simulink model "scheme_L2"  (R2025a)
settings: Solver=ode45  StartTime=0.0  StopTime=12  MaxStep=0.005  RelTol=1e-9  AbsTol=1e-11
settings Model: Creator=dmitriy-nkv  LastModifiedBy=dmitriy-nkv

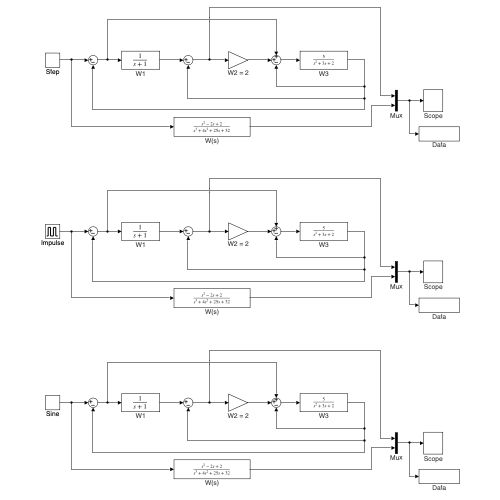
[thumbnail: Simulink's stored preview of the top-level diagram]
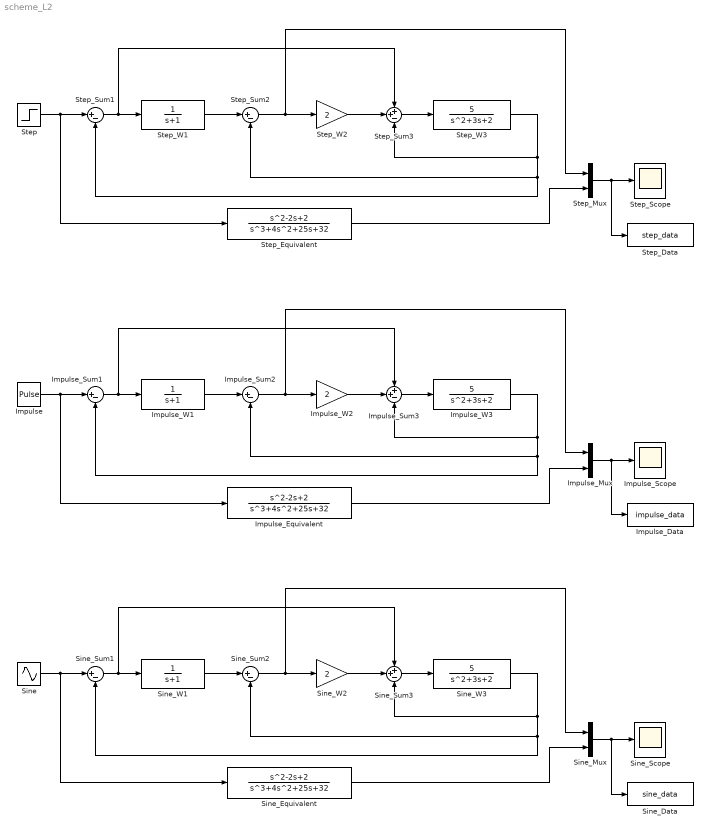
== system scheme_L2 ==
  Impulse : DiscretePulseGenerator  PulseType=Time based  Amplitude=100  Period=20  PulseWidth=0.05  PhaseDelay=1
  Impulse_Data : ToWorkspace  VariableName=impulse_data  SaveFormat=Timeseries  SampleTime=-1
      settings: AttributesFormatString=Data
  Impulse_Equivalent : TransferFcn  Numerator=[1 -2 2]  Denominator=[1 4 25 32]
      settings: AttributesFormatString=W(s)
  Impulse_Mux : Mux  Inputs=2
      settings: AttributesFormatString=Mux
  Impulse_Scope : Scope
      settings: AttributesFormatString=Scope  TimeSpan=12
  Impulse_Sum1 : Sum  Inputs=|+-
  Impulse_Sum2 : Sum  Inputs=|+-
  Impulse_Sum3 : Sum  Inputs=++-
  Impulse_W1 : TransferFcn  Denominator=[1 1]
      settings: AttributesFormatString=W1
  Impulse_W2 : Gain  Gain=2
      settings: AttributesFormatString=W2 = 2
  Impulse_W3 : TransferFcn  Numerator=[5]  Denominator=[1 3 2]
      settings: AttributesFormatString=W3
  Sine : Sin  SampleTime=0
  Sine_Data : ToWorkspace  VariableName=sine_data  SaveFormat=Timeseries  SampleTime=-1
      settings: AttributesFormatString=Data
  Sine_Equivalent : TransferFcn  Numerator=[1 -2 2]  Denominator=[1 4 25 32]
      settings: AttributesFormatString=W(s)
  Sine_Mux : Mux  Inputs=2
      settings: AttributesFormatString=Mux
  Sine_Scope : Scope
      settings: AttributesFormatString=Scope  TimeSpan=12
  Sine_Sum1 : Sum  Inputs=|+-
  Sine_Sum2 : Sum  Inputs=|+-
  Sine_Sum3 : Sum  Inputs=++-
  Sine_W1 : TransferFcn  Denominator=[1 1]
      settings: AttributesFormatString=W1
  Sine_W2 : Gain  Gain=2
      settings: AttributesFormatString=W2 = 2
  Sine_W3 : TransferFcn  Numerator=[5]  Denominator=[1 3 2]
      settings: AttributesFormatString=W3
  Step : Step  SampleTime=0
  Step_Data : ToWorkspace  VariableName=step_data  SaveFormat=Timeseries  SampleTime=-1
      settings: AttributesFormatString=Data
  Step_Equivalent : TransferFcn  Numerator=[1 -2 2]  Denominator=[1 4 25 32]
      settings: AttributesFormatString=W(s)
  Step_Mux : Mux  Inputs=2
      settings: AttributesFormatString=Mux
  Step_Scope : Scope
      settings: AttributesFormatString=Scope  TimeSpan=12
  Step_Sum1 : Sum  Inputs=|+-
  Step_Sum2 : Sum  Inputs=|+-
  Step_Sum3 : Sum  Inputs=++-
  Step_W1 : TransferFcn  Denominator=[1 1]
      settings: AttributesFormatString=W1
  Step_W2 : Gain  Gain=2
      settings: AttributesFormatString=W2 = 2
  Step_W3 : TransferFcn  Numerator=[5]  Denominator=[1 3 2]
      settings: AttributesFormatString=W3
  wires:
  Step/1 -> Step_Sum1/1, Step_Equivalent/1
  Step_Sum1/1 -> Step_W1/1, Step_Sum3/1
  Step_W1/1 -> Step_Sum2/1
  Step_Sum2/1 -> Step_W2/1, Step_Mux/1
  Step_W2/1 -> Step_Sum3/2
  Step_Sum3/1 -> Step_W3/1
  Step_W3/1 -> Step_Sum3/3, Step_Sum1/2, Step_Sum2/2
  Step_Equivalent/1 -> Step_Mux/2
  Step_Mux/1 -> Step_Scope/1, Step_Data/1
  Impulse/1 -> Impulse_Sum1/1, Impulse_Equivalent/1
  Impulse_Sum1/1 -> Impulse_W1/1, Impulse_Sum3/1
  Impulse_W1/1 -> Impulse_Sum2/1
  Impulse_Sum2/1 -> Impulse_W2/1, Impulse_Mux/1
  Impulse_W2/1 -> Impulse_Sum3/2
  Impulse_Sum3/1 -> Impulse_W3/1
  Impulse_W3/1 -> Impulse_Sum3/3, Impulse_Sum1/2, Impulse_Sum2/2
  Impulse_Equivalent/1 -> Impulse_Mux/2
  Impulse_Mux/1 -> Impulse_Scope/1, Impulse_Data/1
  Sine/1 -> Sine_Sum1/1, Sine_Equivalent/1
  Sine_Sum1/1 -> Sine_W1/1, Sine_Sum3/1
  Sine_W1/1 -> Sine_Sum2/1
  Sine_Sum2/1 -> Sine_W2/1, Sine_Mux/1
  Sine_W2/1 -> Sine_Sum3/2
  Sine_Sum3/1 -> Sine_W3/1
  Sine_W3/1 -> Sine_Sum3/3, Sine_Sum1/2, Sine_Sum2/2
  Sine_Equivalent/1 -> Sine_Mux/2
  Sine_Mux/1 -> Sine_Scope/1, Sine_Data/1
